simulink model "SoC_Target"  (R2026b)
settings: Solver=FixedStepDiscrete  StopTime=144000  FixedStep=0.01  EnableMultiTasking=on
settings Model: Creator=gdonati  LastModifiedBy=mgado
settings SolverCC: PositivePriorityOrder=on
settings OptimizationCC: DifferentSizesBufferReuse=on  EfficientTunableParamExpr=on  EnhancedBackFolding=on  MaxStackSize=200000  OptimizationCustomize=off  OptimizeBlockOrder=speed  PassReuseOutputArgsAs=Individual arguments  RemoveInternalMemoryZeroInit=on  RemoveRootLevelIOMemoryZeroInit=on
settings DebuggingCC: ParameterTunabilityLossMsg=error
settings HardwareCC: ProdHWDeviceType=ARM Compatible->ARM Cortex-A (64-bit)  ProdLargestAtomicFloat=Double  ProdLargestAtomicInteger=LongLong  ProdLongLongMode=on
settings RTWCC: BuildConfiguration=Faster Runs  Description=Embedded Coder  GPUComputeCapability=5.0  HardwareBoard=Raspberry Pi (64bit)  SystemTargetFile=ert.tlc  TLCOptions="-aInlineSetEventsForThisBaseRateFcn=TLC_FALSE -aSuppressMultiTaskScheduler=TLC_FALSE  -aRateBasedStepFcn=0"  TemplateMakefile=ert_default_tmf  Toolchain=GNU GCC RPIUtils
settings CodeAppCC: ForceParamTrailComments=on  IgnoreCustomStorageClasses=off  InsertBlockDesc=on  OperatorAnnotations=on  SFDataObjDesc=on  SimulinkDataObjDesc=on
settings ERTTargetCC: CodeReplacementLibrary=ARM Cortex-A CMSIS  ExtModeIntrfLevel=Level2 - Open  ExtModeMexFile=ext_xcp  ExtModeStaticAlloc=on  SupportVariableSizeSignals=on

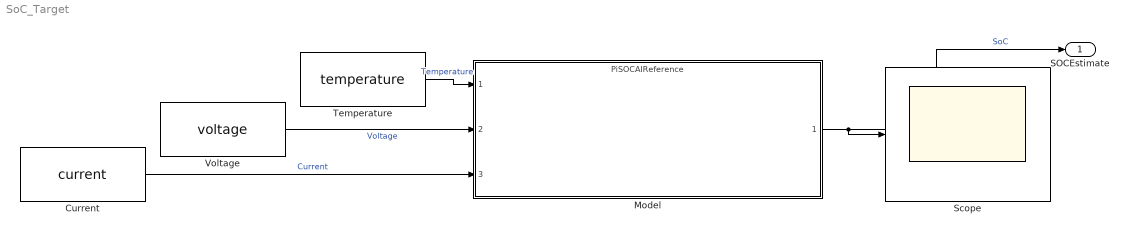
== system SoC_Target ==
  Current : FromWorkspace  VariableName=current  SampleTime=1
  Model : ModelReference  ModelNameDialog=PiSOCAIReference  SimulationMode=Normal  ModelReferenceVersion=1.1
  Scope : Scope
      settings: ActiveDisplayYMinimum=0.46580697740335042  ActiveDisplayYMaximum=0.56614353713712939
  Temperature : FromWorkspace  VariableName=temperature  SampleTime=1
  Voltage : FromWorkspace  VariableName=voltage  SampleTime=1
  SOCEstimate : Outport
  wires:
  Voltage/1 -> Model/2  "Voltage"
  Temperature/1 -> Model/1  "Temperature"
  Current/1 -> Model/3  "Current"
  Model/1 -> Scope/1, SOCEstimate/1  "SoC"
